simulink model "mars_rover_test_harness_chassis"  (R2025a)
settings: Solver=ode23t  StartTime=0.0  StopTime=30  FixedStep=1e-10  MaxStep=1e-1  RelTol=1e-3  AbsTol=1e-3  EnableMultiTasking=on
undefined symbols (not defined in the file): arm_q0, Control, L1, L2, L3, LS1, LS3, R1, R2, R3, Rover, RS1, RS3, X, Y, Z
libraries: sm_lib x119, nesl_utility x99, fl_lib x85, sdl_lib x20, ee_lib x10, mars_rover_lib x8, simulink x5, slpidlib x3, batteryecm_lib x2
(part 6 of 8)

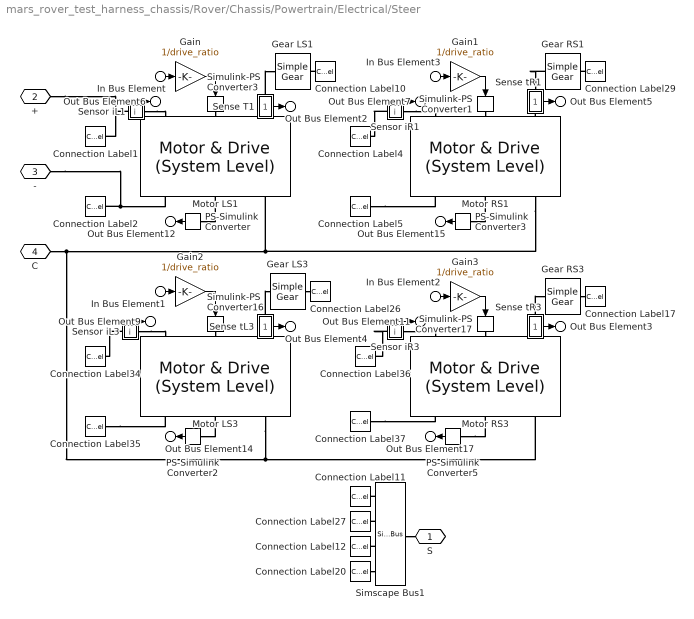
== system mars_rover_test_harness_chassis/Rover/Chassis/Powertrain/Electrical/Steer ==
  In Bus Element : Inport  PortName=Trq  Element=trq.L1
  In Bus Element1 : Inport  PortName=Trq  Element=trq.L3
  In Bus Element2 : Inport  PortName=Trq  Element=trq.R3
  In Bus Element3 : Inport  PortName=Trq  Element=trq.R1
  Connection Label{1,4,34,36} (4 alike) : ConnectionLabel  Label=p
  Connection Label10 : ConnectionLabel  Label=LS1
  Connection Label11 : ConnectionLabel  Label=LS1
  Connection Label12 : ConnectionLabel  Label=RS1
  Connection Label17 : ConnectionLabel  Label=RS3
  Connection Label{2,5,35,37} (4 alike) : ConnectionLabel  Label=n
  Connection Label20 : ConnectionLabel  Label=RS3
  Connection Label26 : ConnectionLabel  Label=LS3
  Connection Label27 : ConnectionLabel  Label=LS3
  Connection Label29 : ConnectionLabel  Label=RS1
  Gain{,1..3} (4 alike) : Gain  Gain=1/drive_ratio
  Gear LS3 : sdl_lib/Gears/Simple Gear  ratio=drive_ratio  rotation_direction=sdl.enum.shaftOutputDirection.same  friction_model=sdl.enum.gear_efficiencies_load.off  T_noload=0.1 N*m  T_nom=5 N*m  efficiency_nom=0.8  efficiency=drive_efficiency  temperature_TLU=[280, 300, 320] K  load_TLU=[1, 5, 10] N*m  efficiency_TLU=[.95, .9, .85]  efficiency_TLU2=[.85, .8, .75; .95, .9, .85; .85, .8, .7]  w_thr=0.01 rad/s  pwr_thr=0.001 W  enable_backlash=false  hardstop_model=simscape.enum.hardstop.smooth  backlash_distance=1e-3 mm  r_base=0.1 m  transition=1e-4 mm  backlash_stiffness=1e7 N/m  backlash_damping=1e6 N/(m/s)  coeff_rest=0  v_tol=0.001 m/s  f_tol=0 N  mu_visc=[0, 0] N*m/(rad/s)  thermal_mass=50 J/K  temperature_specify=off  temperature_priority=High  temperature=300 K  temperature_nominal_specify=off  temperature_nominal_value=1  temperature_nominal_unit=K  x_backlash_specify=off  x_backlash_priority=None  x_backlash=0 mm  x_backlash_nominal_specify=off  x_backlash_nominal_value=1  x_backlash_nominal_unit=mm  f_hardstop_specify=off  f_hardstop_priority=None  f_hardstop=0 N  f_hardstop_nominal_specify=off  f_hardstop_nominal_value=1  f_hardstop_nominal_unit=N  v_backlash_specify=off  v_backlash_priority=None  v_backlash=0 m/s  v_backlash_nominal_specify=off  v_backlash_nominal_value=1  v_backlash_nominal_unit=m/s
  Gear RS1 : sdl_lib/Gears/Simple Gear  ratio=drive_ratio  rotation_direction=sdl.enum.shaftOutputDirection.same  friction_model=sdl.enum.gear_efficiencies_load.off  T_noload=0.1 N*m  T_nom=5 N*m  efficiency_nom=0.8  efficiency=drive_efficiency  temperature_TLU=[280, 300, 320] K  load_TLU=[1, 5, 10] N*m  efficiency_TLU=[.95, .9, .85]  efficiency_TLU2=[.85, .8, .75; .95, .9, .85; .85, .8, .7]  w_thr=0.01 rad/s  pwr_thr=0.001 W  enable_backlash=false  hardstop_model=simscape.enum.hardstop.smooth  backlash_distance=1e-3 mm  r_base=0.1 m  transition=1e-4 mm  backlash_stiffness=1e7 N/m  backlash_damping=1e6 N/(m/s)  coeff_rest=0  v_tol=0.001 m/s  f_tol=0 N  mu_visc=[0, 0] N*m/(rad/s)  thermal_mass=50 J/K  temperature_specify=off  temperature_priority=High  temperature=300 K  temperature_nominal_specify=off  temperature_nominal_value=1  temperature_nominal_unit=K  x_backlash_specify=off  x_backlash_priority=None  x_backlash=0 mm  x_backlash_nominal_specify=off  x_backlash_nominal_value=1  x_backlash_nominal_unit=mm  f_hardstop_specify=off  f_hardstop_priority=None  f_hardstop=0 N  f_hardstop_nominal_specify=off  f_hardstop_nominal_value=1  f_hardstop_nominal_unit=N  v_backlash_specify=off  v_backlash_priority=None  v_backlash=0 m/s  v_backlash_nominal_specify=off  v_backlash_nominal_value=1  v_backlash_nominal_unit=m/s
  Gear RS3 : sdl_lib/Gears/Simple Gear  ratio=drive_ratio  rotation_direction=sdl.enum.shaftOutputDirection.same  friction_model=sdl.enum.gear_efficiencies_load.off  T_noload=0.1 N*m  T_nom=5 N*m  efficiency_nom=0.8  efficiency=drive_efficiency  temperature_TLU=[280, 300, 320] K  load_TLU=[1, 5, 10] N*m  efficiency_TLU=[.95, .9, .85]  efficiency_TLU2=[.85, .8, .75; .95, .9, .85; .85, .8, .7]  w_thr=0.01 rad/s  pwr_thr=0.001 W  enable_backlash=false  hardstop_model=simscape.enum.hardstop.smooth  backlash_distance=1e-3 mm  r_base=0.1 m  transition=1e-4 mm  backlash_stiffness=1e7 N/m  backlash_damping=1e6 N/(m/s)  coeff_rest=0  v_tol=0.001 m/s  f_tol=0 N  mu_visc=[0, 0] N*m/(rad/s)  thermal_mass=50 J/K  temperature_specify=off  temperature_priority=High  temperature=300 K  temperature_nominal_specify=off  temperature_nominal_value=1  temperature_nominal_unit=K  x_backlash_specify=off  x_backlash_priority=None  x_backlash=0 mm  x_backlash_nominal_specify=off  x_backlash_nominal_value=1  x_backlash_nominal_unit=mm  f_hardstop_specify=off  f_hardstop_priority=None  f_hardstop=0 N  f_hardstop_nominal_specify=off  f_hardstop_nominal_value=1  f_hardstop_nominal_unit=N  v_backlash_specify=off  v_backlash_priority=None  v_backlash=0 m/s  v_backlash_nominal_specify=off  v_backlash_nominal_value=1  v_backlash_nominal_unit=m/s
  Gear LS1 : sdl_lib/Gears/Simple Gear  ratio=drive_ratio  rotation_direction=sdl.enum.shaftOutputDirection.same  friction_model=sdl.enum.gear_efficiencies_load.off  T_noload=0.1 N*m  T_nom=5 N*m  efficiency_nom=0.8  efficiency=drive_efficiency  temperature_TLU=[280, 300, 320] K  load_TLU=[1, 5, 10] N*m  efficiency_TLU=[.95, .9, .85]  efficiency_TLU2=[.85, .8, .75; .95, .9, .85; .85, .8, .7]  w_thr=0.01 rad/s  pwr_thr=0.001 W  enable_backlash=false  hardstop_model=simscape.enum.hardstop.smooth  backlash_distance=1e-3 mm  r_base=0.1 m  transition=1e-4 mm  backlash_stiffness=1e7 N/m  backlash_damping=1e6 N/(m/s)  coeff_rest=0  v_tol=0.001 m/s  f_tol=0 N  mu_visc=[0, 0] N*m/(rad/s)  thermal_mass=50 J/K  temperature_specify=off  temperature_priority=High  temperature=300 K  temperature_nominal_specify=off  temperature_nominal_value=1  temperature_nominal_unit=K  x_backlash_specify=off  x_backlash_priority=None  x_backlash=0 mm  x_backlash_nominal_specify=off  x_backlash_nominal_value=1  x_backlash_nominal_unit=mm  f_hardstop_specify=off  f_hardstop_priority=None  f_hardstop=0 N  f_hardstop_nominal_specify=off  f_hardstop_nominal_value=1  f_hardstop_nominal_unit=N  v_backlash_specify=off  v_backlash_priority=None  v_backlash=0 m/s  v_backlash_nominal_specify=off  v_backlash_nominal_value=1  v_backlash_nominal_unit=m/s
  Motor LS1 : ee_lib/Electromechanical/Motor & Drive (System Level)  torque_speed_param=ee.enum.electromech.envelope.torque_power  overtorque_param=ee.enum.electromech.overtorque.no  T_t=[.09, .08, .07, 0] N*m  T_t_intermittent=[.36, .32, .28, 0] N*m  T_t_2D=[.09, .09, .09; .08, .08, .08; .07, .07, .07; 0, 0, 0] N*m  T_t_intermittent_2D=[.36, .36, .36; .32, .32, .32; .28, .28, .28; 0, 0, 0] N*m  w_t=[0, 3750, 7500, 8000] rpm  vdc_t=[6, 12, 24] V  torque_max=trq_max N*m  power_max=power_max W  torque_max_intermittent=0.4 N*m  power_max_intermittent=120 W  time_overtorque=30 s  time_recover=60 s  Tc=trq_tc s  EnableSwitch=simscape.enum.onoff.off  losses_param=1  eff=eff_overall  w_eff=eff_spd rpm  T_eff=eff_trq N*m  Piron=0 % not important in first iteration W  Pbase=0 % not important in first iteration W  w_eff_vec=[-8000, -4000, 0, 4000, 8000] rpm  T_eff_vec=[0, .03, .06, .09] N*m  v_eff_vec=[100, 250, 400] V  losses_mat=[1.49, 1.67, 2.21, 3.1; .42, .69, 1.14, 2.03; .06, .24, .78, 1.68; .42, .69, 1.14, 2.03; 1.49, 1.67, 2.21, 3.1] W  efficiency_mat=[95, 95, 95, 95; 95, 95, 95, 95; 95, 95, 95, 95; 95, 95, 95, 95; 95, 95, 95, 95]  losses_mat_3D=ones(5, 4, 3) W  efficiency_mat_3D=95 * ones(5, 4, 3)  Res=0 % not important in first iteration Ohm  J=0 kg*m^2  lam=rotor_d N*m/(rad/s)  speed0=0 rpm  faulted_specify=off  faulted_priority=None  faulted=0  faulted_nominal_specify=off  faulted_nominal_value=1  faulted_nominal_unit=1  isSwitchedOff_specify=off  isSwitchedOff_priority=None  isSwitchedOff=0  isSwitchedOff_nominal_specify=off  isSwitchedOff_nominal_value=1  isSwitchedOff_nominal_unit=1  torqueLimitContinuous_specify=off  torqueLimitContinuous_priority=None  torqueLimitContinuous=0 N*m  torqueLimitContinuous_nominal_specify=off  torqueLimitContinuous_nominal_value=1  torqueLimitContinuous_nominal_unit=N*m  alpha=3.93e-3 1/K  Tmeas=25 degC  Tmeas2=125 degC  losses_mat_T2=[1.49, 1.74, 2.49, 3.74; .42, .67, 1.42, 2.67; .06, .31, 1.06, 2.31; .42, .67, 1.42, 2.67; 1.49, 1.74, 2.49, 3.74] W  efficiency_mat_T2=[95, 95, 95, 95; 95, 95, 95, 95; 95, 95, 95, 95; 95, 95, 95, 95; 95, 95, 95, 95]  losses_mat_3D_T2=ones(5, 4, 3) W  efficiency_mat_3D_T2=95 * ones(5, 4, 3)  thermal_mass=100 J/K  initial_temperature=25 degC
  Motor LS3 : ee_lib/Electromechanical/Motor & Drive (System Level)  torque_speed_param=ee.enum.electromech.envelope.torque_power  overtorque_param=ee.enum.electromech.overtorque.no  T_t=[.09, .08, .07, 0] N*m  T_t_intermittent=[.36, .32, .28, 0] N*m  T_t_2D=[.09, .09, .09; .08, .08, .08; .07, .07, .07; 0, 0, 0] N*m  T_t_intermittent_2D=[.36, .36, .36; .32, .32, .32; .28, .28, .28; 0, 0, 0] N*m  w_t=[0, 3750, 7500, 8000] rpm  vdc_t=[6, 12, 24] V  torque_max=trq_max N*m  power_max=power_max W  torque_max_intermittent=0.4 N*m  power_max_intermittent=120 W  time_overtorque=30 s  time_recover=60 s  Tc=trq_tc s  EnableSwitch=simscape.enum.onoff.off  losses_param=1  eff=eff_overall  w_eff=eff_spd rpm  T_eff=eff_trq N*m  Piron=0 % not important in first iteration W  Pbase=0 % not important in first iteration W  w_eff_vec=[-8000, -4000, 0, 4000, 8000] rpm  T_eff_vec=[0, .03, .06, .09] N*m  v_eff_vec=[100, 250, 400] V  losses_mat=[1.49, 1.67, 2.21, 3.1; .42, .69, 1.14, 2.03; .06, .24, .78, 1.68; .42, .69, 1.14, 2.03; 1.49, 1.67, 2.21, 3.1] W  efficiency_mat=[95, 95, 95, 95; 95, 95, 95, 95; 95, 95, 95, 95; 95, 95, 95, 95; 95, 95, 95, 95]  losses_mat_3D=ones(5, 4, 3) W  efficiency_mat_3D=95 * ones(5, 4, 3)  Res=0 % not important in first iteration Ohm  J=0 kg*m^2  lam=rotor_d N*m/(rad/s)  speed0=0 rpm  faulted_specify=off  faulted_priority=None  faulted=0  faulted_nominal_specify=off  faulted_nominal_value=1  faulted_nominal_unit=1  isSwitchedOff_specify=off  isSwitchedOff_priority=None  isSwitchedOff=0  isSwitchedOff_nominal_specify=off  isSwitchedOff_nominal_value=1  isSwitchedOff_nominal_unit=1  torqueLimitContinuous_specify=off  torqueLimitContinuous_priority=None  torqueLimitContinuous=0 N*m  torqueLimitContinuous_nominal_specify=off  torqueLimitContinuous_nominal_value=1  torqueLimitContinuous_nominal_unit=N*m  alpha=3.93e-3 1/K  Tmeas=25 degC  Tmeas2=125 degC  losses_mat_T2=[1.49, 1.74, 2.49, 3.74; .42, .67, 1.42, 2.67; .06, .31, 1.06, 2.31; .42, .67, 1.42, 2.67; 1.49, 1.74, 2.49, 3.74] W  efficiency_mat_T2=[95, 95, 95, 95; 95, 95, 95, 95; 95, 95, 95, 95; 95, 95, 95, 95; 95, 95, 95, 95]  losses_mat_3D_T2=ones(5, 4, 3) W  efficiency_mat_3D_T2=95 * ones(5, 4, 3)  thermal_mass=100 J/K  initial_temperature=25 degC
  Motor RS1 : ee_lib/Electromechanical/Motor & Drive (System Level)  torque_speed_param=ee.enum.electromech.envelope.torque_power  overtorque_param=ee.enum.electromech.overtorque.no  T_t=[.09, .08, .07, 0] N*m  T_t_intermittent=[.36, .32, .28, 0] N*m  T_t_2D=[.09, .09, .09; .08, .08, .08; .07, .07, .07; 0, 0, 0] N*m  T_t_intermittent_2D=[.36, .36, .36; .32, .32, .32; .28, .28, .28; 0, 0, 0] N*m  w_t=[0, 3750, 7500, 8000] rpm  vdc_t=[6, 12, 24] V  torque_max=trq_max N*m  power_max=power_max W  torque_max_intermittent=0.4 N*m  power_max_intermittent=120 W  time_overtorque=30 s  time_recover=60 s  Tc=trq_tc s  EnableSwitch=simscape.enum.onoff.off  losses_param=1  eff=eff_overall  w_eff=eff_spd rpm  T_eff=eff_trq N*m  Piron=0 % not important in first iteration W  Pbase=0 % not important in first iteration W  w_eff_vec=[-8000, -4000, 0, 4000, 8000] rpm  T_eff_vec=[0, .03, .06, .09] N*m  v_eff_vec=[100, 250, 400] V  losses_mat=[1.49, 1.67, 2.21, 3.1; .42, .69, 1.14, 2.03; .06, .24, .78, 1.68; .42, .69, 1.14, 2.03; 1.49, 1.67, 2.21, 3.1] W  efficiency_mat=[95, 95, 95, 95; 95, 95, 95, 95; 95, 95, 95, 95; 95, 95, 95, 95; 95, 95, 95, 95]  losses_mat_3D=ones(5, 4, 3) W  efficiency_mat_3D=95 * ones(5, 4, 3)  Res=0 % not important in first iteration Ohm  J=0 kg*m^2  lam=rotor_d N*m/(rad/s)  speed0=0 rpm  faulted_specify=off  faulted_priority=None  faulted=0  faulted_nominal_specify=off  faulted_nominal_value=1  faulted_nominal_unit=1  isSwitchedOff_specify=off  isSwitchedOff_priority=None  isSwitchedOff=0  isSwitchedOff_nominal_specify=off  isSwitchedOff_nominal_value=1  isSwitchedOff_nominal_unit=1  torqueLimitContinuous_specify=off  torqueLimitContinuous_priority=None  torqueLimitContinuous=0 N*m  torqueLimitContinuous_nominal_specify=off  torqueLimitContinuous_nominal_value=1  torqueLimitContinuous_nominal_unit=N*m  alpha=3.93e-3 1/K  Tmeas=25 degC  Tmeas2=125 degC  losses_mat_T2=[1.49, 1.74, 2.49, 3.74; .42, .67, 1.42, 2.67; .06, .31, 1.06, 2.31; .42, .67, 1.42, 2.67; 1.49, 1.74, 2.49, 3.74] W  efficiency_mat_T2=[95, 95, 95, 95; 95, 95, 95, 95; 95, 95, 95, 95; 95, 95, 95, 95; 95, 95, 95, 95]  losses_mat_3D_T2=ones(5, 4, 3) W  efficiency_mat_3D_T2=95 * ones(5, 4, 3)  thermal_mass=100 J/K  initial_temperature=25 degC
  Motor RS3 : ee_lib/Electromechanical/Motor & Drive (System Level)  torque_speed_param=ee.enum.electromech.envelope.torque_power  overtorque_param=ee.enum.electromech.overtorque.no  T_t=[.09, .08, .07, 0] N*m  T_t_intermittent=[.36, .32, .28, 0] N*m  T_t_2D=[.09, .09, .09; .08, .08, .08; .07, .07, .07; 0, 0, 0] N*m  T_t_intermittent_2D=[.36, .36, .36; .32, .32, .32; .28, .28, .28; 0, 0, 0] N*m  w_t=[0, 3750, 7500, 8000] rpm  vdc_t=[6, 12, 24] V  torque_max=trq_max N*m  power_max=power_max W  torque_max_intermittent=0.4 N*m  power_max_intermittent=120 W  time_overtorque=30 s  time_recover=60 s  Tc=trq_tc s  EnableSwitch=simscape.enum.onoff.off  losses_param=1  eff=eff_overall  w_eff=eff_spd rpm  T_eff=eff_trq N*m  Piron=0 % not important in first iteration W  Pbase=0 % not important in first iteration W  w_eff_vec=[-8000, -4000, 0, 4000, 8000] rpm  T_eff_vec=[0, .03, .06, .09] N*m  v_eff_vec=[100, 250, 400] V  losses_mat=[1.49, 1.67, 2.21, 3.1; .42, .69, 1.14, 2.03; .06, .24, .78, 1.68; .42, .69, 1.14, 2.03; 1.49, 1.67, 2.21, 3.1] W  efficiency_mat=[95, 95, 95, 95; 95, 95, 95, 95; 95, 95, 95, 95; 95, 95, 95, 95; 95, 95, 95, 95]  losses_mat_3D=ones(5, 4, 3) W  efficiency_mat_3D=95 * ones(5, 4, 3)  Res=0 % not important in first iteration Ohm  J=0 kg*m^2  lam=rotor_d N*m/(rad/s)  speed0=0 rpm  faulted_specify=off  faulted_priority=None  faulted=0  faulted_nominal_specify=off  faulted_nominal_value=1  faulted_nominal_unit=1  isSwitchedOff_specify=off  isSwitchedOff_priority=None  isSwitchedOff=0  isSwitchedOff_nominal_specify=off  isSwitchedOff_nominal_value=1  isSwitchedOff_nominal_unit=1  torqueLimitContinuous_specify=off  torqueLimitContinuous_priority=None  torqueLimitContinuous=0 N*m  torqueLimitContinuous_nominal_specify=off  torqueLimitContinuous_nominal_value=1  torqueLimitContinuous_nominal_unit=N*m  alpha=3.93e-3 1/K  Tmeas=25 degC  Tmeas2=125 degC  losses_mat_T2=[1.49, 1.74, 2.49, 3.74; .42, .67, 1.42, 2.67; .06, .31, 1.06, 2.31; .42, .67, 1.42, 2.67; 1.49, 1.74, 2.49, 3.74] W  efficiency_mat_T2=[95, 95, 95, 95; 95, 95, 95, 95; 95, 95, 95, 95; 95, 95, 95, 95; 95, 95, 95, 95]  losses_mat_3D_T2=ones(5, 4, 3) W  efficiency_mat_3D_T2=95 * ones(5, 4, 3)  thermal_mass=100 J/K  initial_temperature=25 degC
  PS-Simulink Converter{,2..3,5} (4 alike) : nesl_utility/PS-Simulink Converter  PhysicalDomain=network_engine_domain  SubClassName=ps_output  LeftPortType=input  RightPortType=output  PseudoPeriodic=off  Frequencies=[]  VectorFormat=1-D array  Unit=inherit  AffineConversion=off
  Sense T1 : Subsystem
      settings: PortSchema="{\"entries\":[{\"content\":{\"sides\":[{\"content\":{\"connectorIds\":[\"LConn1\"]},\"type\":\"ConnectorPlacement.EquallySpacedRectSide\",\"uuid\":\"592cc1a1-656f-47ce-ad3a-4b4dc1070b5c\"},{\"content\":{\"connectorIds\":[\"RConn1\"],\"side\":\"RIGHT\"},\"type\":\"ConnectorPlacement.EquallySpacedRectSide\",\"uuid\":\"9bca39c3-eeb4-4456-9b97-61ec2f027d42\"},{\"content\":{\"connectorIds\":[\"Out1\"],\"side\":\"TOP\"},\"type\":\"ConnectorPlacement.EquallySpacedRectSide\",\"uuid\":\"1e04bf27-fb0c-4be4-96d5-7a7c6152a7df\"}]},\"type\":\"ConnectorPlacement.EquallySpacedConnector\",\"uuid\":\"70eba8cc-e966-48e4-a1ce-5ccb9693dc60\"}],\"packageUris\":[\"http://schema.mathworks.com/mf0/Connector/R2020b\"],\"version\":\"1.0\"}"
      mask Display: disp('t')
  Sense tL3 : Subsystem
      settings: PortSchema="{\"entries\":[{\"content\":{\"sides\":[{\"content\":{\"connectorIds\":[\"LConn1\"]},\"type\":\"ConnectorPlacement.EquallySpacedRectSide\",\"uuid\":\"592cc1a1-656f-47ce-ad3a-4b4dc1070b5c\"},{\"content\":{\"connectorIds\":[\"RConn1\"],\"side\":\"RIGHT\"},\"type\":\"ConnectorPlacement.EquallySpacedRectSide\",\"uuid\":\"9bca39c3-eeb4-4456-9b97-61ec2f027d42\"},{\"content\":{\"connectorIds\":[\"Out1\"],\"side\":\"TOP\"},\"type\":\"ConnectorPlacement.EquallySpacedRectSide\",\"uuid\":\"1e04bf27-fb0c-4be4-96d5-7a7c6152a7df\"}]},\"type\":\"ConnectorPlacement.EquallySpacedConnector\",\"uuid\":\"70eba8cc-e966-48e4-a1ce-5ccb9693dc60\"}],\"packageUris\":[\"http://schema.mathworks.com/mf0/Connector/R2020b\"],\"version\":\"1.0\"}"
      mask Display: disp('t')
  Sense tR1 : Subsystem
      settings: PortSchema="{\"entries\":[{\"content\":{\"sides\":[{\"content\":{\"connectorIds\":[\"LConn1\"]},\"type\":\"ConnectorPlacement.EquallySpacedRectSide\",\"uuid\":\"592cc1a1-656f-47ce-ad3a-4b4dc1070b5c\"},{\"content\":{\"connectorIds\":[\"RConn1\"],\"side\":\"RIGHT\"},\"type\":\"ConnectorPlacement.EquallySpacedRectSide\",\"uuid\":\"9bca39c3-eeb4-4456-9b97-61ec2f027d42\"},{\"content\":{\"connectorIds\":[\"Out1\"],\"side\":\"TOP\"},\"type\":\"ConnectorPlacement.EquallySpacedRectSide\",\"uuid\":\"1e04bf27-fb0c-4be4-96d5-7a7c6152a7df\"}]},\"type\":\"ConnectorPlacement.EquallySpacedConnector\",\"uuid\":\"70eba8cc-e966-48e4-a1ce-5ccb9693dc60\"}],\"packageUris\":[\"http://schema.mathworks.com/mf0/Connector/R2020b\"],\"version\":\"1.0\"}"
      mask Display: disp('t')
  Sense tR3 : Subsystem
      settings: PortSchema="{\"entries\":[{\"content\":{\"sides\":[{\"content\":{\"connectorIds\":[\"LConn1\"]},\"type\":\"ConnectorPlacement.EquallySpacedRectSide\",\"uuid\":\"592cc1a1-656f-47ce-ad3a-4b4dc1070b5c\"},{\"content\":{\"connectorIds\":[\"RConn1\"],\"side\":\"RIGHT\"},\"type\":\"ConnectorPlacement.EquallySpacedRectSide\",\"uuid\":\"9bca39c3-eeb4-4456-9b97-61ec2f027d42\"},{\"content\":{\"connectorIds\":[\"Out1\"],\"side\":\"TOP\"},\"type\":\"ConnectorPlacement.EquallySpacedRectSide\",\"uuid\":\"1e04bf27-fb0c-4be4-96d5-7a7c6152a7df\"}]},\"type\":\"ConnectorPlacement.EquallySpacedConnector\",\"uuid\":\"70eba8cc-e966-48e4-a1ce-5ccb9693dc60\"}],\"packageUris\":[\"http://schema.mathworks.com/mf0/Connector/R2020b\"],\"version\":\"1.0\"}"
      mask Display: disp('t')
  Sensor iL1 : Subsystem
      settings: PortSchema="{\"entries\":[{\"content\":{\"sides\":[{\"content\":{\"connectorIds\":[\"LConn1\"]},\"type\":\"ConnectorPlacement.EquallySpacedRectSide\",\"uuid\":\"592cc1a1-656f-47ce-ad3a-4b4dc1070b5c\"},{\"content\":{\"connectorIds\":[\"RConn1\"],\"side\":\"RIGHT\"},\"type\":\"ConnectorPlacement.EquallySpacedRectSide\",\"uuid\":\"9bca39c3-eeb4-4456-9b97-61ec2f027d42\"},{\"content\":{\"connectorIds\":[\"Out1\"],\"side\":\"TOP\"},\"type\":\"ConnectorPlacement.EquallySpacedRectSide\",\"uuid\":\"1e04bf27-fb0c-4be4-96d5-7a7c6152a7df\"}]},\"type\":\"ConnectorPlacement.EquallySpacedConnector\",\"uuid\":\"70eba8cc-e966-48e4-a1ce-5ccb9693dc60\"}],\"packageUris\":[\"http://schema.mathworks.com/mf0/Connector/R2020b\"],\"version\":\"1.0\"}"
      mask Display: disp('i');
  Sensor iL3 : Subsystem
      settings: PortSchema="{\"entries\":[{\"content\":{\"sides\":[{\"content\":{\"connectorIds\":[\"LConn1\"]},\"type\":\"ConnectorPlacement.EquallySpacedRectSide\",\"uuid\":\"592cc1a1-656f-47ce-ad3a-4b4dc1070b5c\"},{\"content\":{\"connectorIds\":[\"RConn1\"],\"side\":\"RIGHT\"},\"type\":\"ConnectorPlacement.EquallySpacedRectSide\",\"uuid\":\"9bca39c3-eeb4-4456-9b97-61ec2f027d42\"},{\"content\":{\"connectorIds\":[\"Out1\"],\"side\":\"TOP\"},\"type\":\"ConnectorPlacement.EquallySpacedRectSide\",\"uuid\":\"1e04bf27-fb0c-4be4-96d5-7a7c6152a7df\"}]},\"type\":\"ConnectorPlacement.EquallySpacedConnector\",\"uuid\":\"70eba8cc-e966-48e4-a1ce-5ccb9693dc60\"}],\"packageUris\":[\"http://schema.mathworks.com/mf0/Connector/R2020b\"],\"version\":\"1.0\"}"
      mask Display: disp('i');
  Sensor iR1 : Subsystem
      settings: PortSchema="{\"entries\":[{\"content\":{\"sides\":[{\"content\":{\"connectorIds\":[\"LConn1\"]},\"type\":\"ConnectorPlacement.EquallySpacedRectSide\",\"uuid\":\"592cc1a1-656f-47ce-ad3a-4b4dc1070b5c\"},{\"content\":{\"connectorIds\":[\"RConn1\"],\"side\":\"RIGHT\"},\"type\":\"ConnectorPlacement.EquallySpacedRectSide\",\"uuid\":\"9bca39c3-eeb4-4456-9b97-61ec2f027d42\"},{\"content\":{\"connectorIds\":[\"Out1\"],\"side\":\"TOP\"},\"type\":\"ConnectorPlacement.EquallySpacedRectSide\",\"uuid\":\"1e04bf27-fb0c-4be4-96d5-7a7c6152a7df\"}]},\"type\":\"ConnectorPlacement.EquallySpacedConnector\",\"uuid\":\"70eba8cc-e966-48e4-a1ce-5ccb9693dc60\"}],\"packageUris\":[\"http://schema.mathworks.com/mf0/Connector/R2020b\"],\"version\":\"1.0\"}"
      mask Display: disp('i');
  Sensor iR3 : Subsystem
      settings: PortSchema="{\"entries\":[{\"content\":{\"sides\":[{\"content\":{\"connectorIds\":[\"LConn1\"]},\"type\":\"ConnectorPlacement.EquallySpacedRectSide\",\"uuid\":\"592cc1a1-656f-47ce-ad3a-4b4dc1070b5c\"},{\"content\":{\"connectorIds\":[\"RConn1\"],\"side\":\"RIGHT\"},\"type\":\"ConnectorPlacement.EquallySpacedRectSide\",\"uuid\":\"9bca39c3-eeb4-4456-9b97-61ec2f027d42\"},{\"content\":{\"connectorIds\":[\"Out1\"],\"side\":\"TOP\"},\"type\":\"ConnectorPlacement.EquallySpacedRectSide\",\"uuid\":\"1e04bf27-fb0c-4be4-96d5-7a7c6152a7df\"}]},\"type\":\"ConnectorPlacement.EquallySpacedConnector\",\"uuid\":\"70eba8cc-e966-48e4-a1ce-5ccb9693dc60\"}],\"packageUris\":[\"http://schema.mathworks.com/mf0/Connector/R2020b\"],\"version\":\"1.0\"}"
      mask Display: disp('i');
  Simscape Bus1 : SimscapeBus  HierarchyStrings=LS1;LS3;RS1;RS3
  Simulink-PS Converter{1,3,16..17} (4 alike) : nesl_utility/Simulink-PS Converter  PhysicalDomain=network_engine_domain  SubClassName=ps_input  LeftPortType=input  RightPortType=output  PseudoPeriodic=off  Frequencies=[]  NoiseDistribution=none  NoiseParameters=[]  Unit=N*m  AffineConversion=off  FilteringAndDerivatives=provide  SimscapeFilterOrder=1  InputFilterTimeConstant=0.001  UdotUserProvided=0
  S : PMIOPort  Side=Right
  + : PMIOPort  Port=2  Side=Left
  - : PMIOPort  Port=3  Side=Left
  C : PMIOPort  Port=4  Side=Right
  Out Bus Element2 : Outport  PortName=m  Element=trq.L1
  Out Bus Element4 : Outport  PortName=m  Element=trq.L3
  Out Bus Element5 : Outport  PortName=m  Element=trq.R1
  Out Bus Element3 : Outport  PortName=m  Element=trq.R3
  Out Bus Element11 : Outport  PortName=m  Element=i.R3
  Out Bus Element6 : Outport  PortName=m  Element=i.L1
  Out Bus Element9 : Outport  PortName=m  Element=i.L3
  Out Bus Element7 : Outport  PortName=m  Element=i.R1
  Out Bus Element12 : Outport  PortName=m  Element=w.L1
  Out Bus Element14 : Outport  PortName=m  Element=w.L3
  Out Bus Element15 : Outport  PortName=m  Element=w.R1
  Out Bus Element17 : Outport  PortName=m  Element=w.R3
  wires:
  Gain2/1 -> Simulink-PS Converter16/1
  In Bus Element2/1 -> Gain3/1
  In Bus Element3/1 -> Gain1/1
  In Bus Element/1 -> Gain/1
  Gain/1 -> Simulink-PS Converter3/1
  Gain1/1 -> Simulink-PS Converter1/1
  In Bus Element1/1 -> Gain2/1
  Gain3/1 -> Simulink-PS Converter17/1
  PS-Simulink Converter/1 -> Out Bus Element12/1
  Sensor iL3/1(i) -> Out Bus Element9/1
  Sense tR3/1(T) -> Out Bus Element3/1
  Sensor iR3/1(i) -> Out Bus Element11/1
  Sensor iR1/1(i) -> Out Bus Element7/1
  Sensor iL1/1(i) -> Out Bus Element6/1
  Sense tL3/1(T) -> Out Bus Element4/1
  Sense T1/1(T) -> Out Bus Element2/1
  PS-Simulink Converter5/1 -> Out Bus Element17/1
  Sense tR1/1(T) -> Out Bus Element5/1
  PS-Simulink Converter3/1 -> Out Bus Element15/1
  PS-Simulink Converter2/1 -> Out Bus Element14/1
  connections:
  Sensor iR1/RConn1 -- Motor RS1/LConn1
  Sensor iR1/LConn1 -- Connection Label4/LConn1
  Simscape Bus1/RConn1 -- S/RConn1
  Connection Label5/LConn1 -- Motor RS1/RConn1
  Motor RS1/RConn3 -- Motor LS1/RConn3 -- C/RConn1 -- Motor LS3/RConn3 -- Motor RS3/RConn3
  Connection Label37/LConn1 -- Motor RS3/RConn1
  Simulink-PS Converter3/RConn1 -- Motor LS1/LConn2
  Simulink-PS Converter16/RConn1 -- Motor LS3/LConn2
  Sensor iL3/LConn1 -- Connection Label34/LConn1
  Connection Label29/LConn1 -- Gear RS1/RConn1
  Simscape Bus1/LConn1 -- Connection Label11/LConn1
  Simulink-PS Converter17/RConn1 -- Motor RS3/LConn2
  Simscape Bus1/LConn3 -- Connection Label12/LConn1
  Simulink-PS Converter1/RConn1 -- Motor RS1/LConn2
  Simscape Bus1/LConn2 -- Connection Label27/LConn1
  Sensor iR3/RConn1 -- Motor RS3/LConn1
  Sensor iL1/RConn1 -- Motor LS1/LConn1
  Sensor iR3/LConn1 -- Connection Label36/LConn1
  PS-Simulink Converter2/LConn1 -- Motor LS3/RConn2
  Connection Label35/LConn1 -- Motor LS3/RConn1
  Sensor iL3/RConn1 -- Motor LS3/LConn1
  Connection Label20/LConn1 -- Simscape Bus1/LConn4
  PS-Simulink Converter5/LConn1 -- Motor RS3/RConn2
  PS-Simulink Converter/LConn1 -- Motor LS1/RConn2
  PS-Simulink Converter3/LConn1 -- Motor RS1/RConn2
  +/RConn1 -- Sensor iL1/LConn1 -- Connection Label1/LConn1
  -/RConn1 -- Motor LS1/RConn1 -- Connection Label2/LConn1
  Connection Label10/LConn1 -- Gear LS1/RConn1
  Gear LS3/RConn1 -- Connection Label26/LConn1
  Gear RS3/RConn1 -- Connection Label17/LConn1
  Sense T1/LConn1 -- Gear LS1/LConn1
  Sense T1/RConn1 -- Motor LS1/LConn3
  Motor RS1/LConn3 -- Sense tR1/RConn1
  Gear RS1/LConn1 -- Sense tR1/LConn1
  Sense tL3/LConn1 -- Gear LS3/LConn1
  Sense tL3/RConn1 -- Motor LS3/LConn3
  Sense tR3/LConn1 -- Gear RS3/LConn1
  Motor RS3/LConn3 -- Sense tR3/RConn1

== system mars_rover_test_harness_chassis/Rover/Chassis/Powertrain/Ideal/Calculate Power ==
  S : Inport
  D : Inport  Port=2
  Abs : Abs  ZeroCross=off  SaturateOnIntegerOverflow=off
  Bus Selector : BusSelector  OutputSignals=w.L1,trq.L1,w.L3,trq.L3,w.R1,trq.R1,w.R3,trq.R3
  Bus Selector1 : BusSelector  OutputSignals=w.L1,trq.L1,w.L2,trq.L2,w.L3,trq.L3,w.R1,trq.R1,w.R2,trq.R2,w.R3,trq.R3
  Product{,1..9} (10 alike) : Product
  R : Gain  Gain=1/100
  Sum : Sum  Inputs=++++
  Sum1 : Sum  Inputs=++++++
  Sum2 : Sum
  i : Outport
  wires:
  S/1 -> Bus Selector/1
  Bus Selector/1 -> Product/1  "<L1>"
  Bus Selector/2 -> Product/2  "<L1>"
  Bus Selector/3 -> Product1/1  "<L3>"
  Bus Selector/4 -> Product1/2  "<L3>"
  Bus Selector/6 -> Product2/2  "<R1>"
  Bus Selector/5 -> Product2/1  "<R1>"
  Product/1 -> Sum/1
  Product1/1 -> Sum/2
  Product2/1 -> Sum/3
  Product3/1 -> Sum/4
  D/1 -> Bus Selector1/1
  Product7/1 -> Sum1/4
  Product6/1 -> Sum1/3
  Product5/1 -> Sum1/2
  Product4/1 -> Sum1/1
  Bus Selector1/1 -> Product4/1  "<L1>"
  Bus Selector1/2 -> Product4/2  "<L1>"
  Product8/1 -> Sum1/5
  Product9/1 -> Sum1/6
  Bus Selector1/3 -> Product5/1  "<L2>"
  Bus Selector1/4 -> Product5/2  "<L2>"
  Bus Selector1/5 -> Product6/1  "<L3>"
  Bus Selector1/6 -> Product6/2  "<L3>"
  Bus Selector1/7 -> Product7/1  "<R1>"
  Bus Selector1/8 -> Product7/2  "<R1>"
  Bus Selector1/9 -> Product8/1  "<R2>"
  Bus Selector1/10 -> Product8/2  "<R2>"
  Bus Selector1/11 -> Product9/1  "<R3>"
  Bus Selector1/12 -> Product9/2  "<R3>"
  Sum1/1 -> Sum2/2
  Sum/1 -> Sum2/1
  Sum2/1 -> Abs/1
  Abs/1 -> R/1
  Bus Selector/7 -> Product3/1  "<R3>"
  Bus Selector/8 -> Product3/2  "<R3>"
  R/1 -> i/1

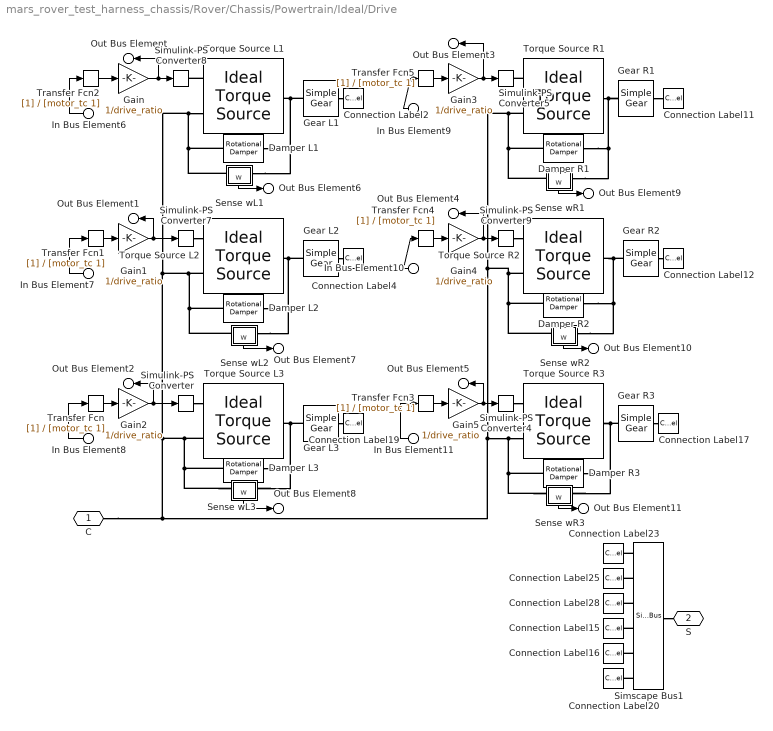
== system mars_rover_test_harness_chassis/Rover/Chassis/Powertrain/Ideal/Drive ==
  In Bus Element6 : Inport  PortName=Trq  Element=trq.L1
  In Bus Element7 : Inport  PortName=Trq  Element=trq.L2
  In Bus Element8 : Inport  PortName=Trq  Element=trq.L3
  In Bus Element9 : Inport  PortName=Trq  Element=trq.R1
  In Bus Element10 : Inport  PortName=Trq  Element=trq.R2
  In Bus Element11 : Inport  PortName=Trq  Element=trq.R3
  Connection Label11 : ConnectionLabel  Label=R1
  Connection Label12 : ConnectionLabel  Label=R2
  Connection Label15 : ConnectionLabel  Label=R1
  Connection Label16 : ConnectionLabel  Label=R2
  Connection Label17 : ConnectionLabel  Label=R3
  Connection Label19 : ConnectionLabel  Label=L3
  Connection Label2 : ConnectionLabel  Label=L1
  Connection Label20 : ConnectionLabel  Label=R3
  Connection Label23 : ConnectionLabel  Label=L1
  Connection Label25 : ConnectionLabel  Label=L2
  Connection Label28 : ConnectionLabel  Label=L3
  Connection Label4 : ConnectionLabel  Label=L2
  Damper L1 : fl_lib/Mechanical/Rotational Elements/Rotational Damper  D=motor_d N*m/(rad/s)  w_specify=off  w_priority=None  w=0 rad/s  w_nominal_specify=off  w_nominal_value=1  w_nominal_unit=rad/s  t_specify=off  t_priority=None  t=0 N*m  t_nominal_specify=off  t_nominal_value=1  t_nominal_unit=N*m
  Damper L2 : fl_lib/Mechanical/Rotational Elements/Rotational Damper  D=motor_d N*m/(rad/s)  w_specify=off  w_priority=None  w=0 rad/s  w_nominal_specify=off  w_nominal_value=1  w_nominal_unit=rad/s  t_specify=off  t_priority=None  t=0 N*m  t_nominal_specify=off  t_nominal_value=1  t_nominal_unit=N*m
  Damper L3 : fl_lib/Mechanical/Rotational Elements/Rotational Damper  D=motor_d N*m/(rad/s)  w_specify=off  w_priority=None  w=0 rad/s  w_nominal_specify=off  w_nominal_value=1  w_nominal_unit=rad/s  t_specify=off  t_priority=None  t=0 N*m  t_nominal_specify=off  t_nominal_value=1  t_nominal_unit=N*m
  Damper R1 : fl_lib/Mechanical/Rotational Elements/Rotational Damper  D=motor_d N*m/(rad/s)  w_specify=off  w_priority=None  w=0 rad/s  w_nominal_specify=off  w_nominal_value=1  w_nominal_unit=rad/s  t_specify=off  t_priority=None  t=0 N*m  t_nominal_specify=off  t_nominal_value=1  t_nominal_unit=N*m
  Damper R2 : fl_lib/Mechanical/Rotational Elements/Rotational Damper  D=motor_d N*m/(rad/s)  w_specify=off  w_priority=None  w=0 rad/s  w_nominal_specify=off  w_nominal_value=1  w_nominal_unit=rad/s  t_specify=off  t_priority=None  t=0 N*m  t_nominal_specify=off  t_nominal_value=1  t_nominal_unit=N*m
  Damper R3 : fl_lib/Mechanical/Rotational Elements/Rotational Damper  D=motor_d N*m/(rad/s)  w_specify=off  w_priority=None  w=0 rad/s  w_nominal_specify=off  w_nominal_value=1  w_nominal_unit=rad/s  t_specify=off  t_priority=None  t=0 N*m  t_nominal_specify=off  t_nominal_value=1  t_nominal_unit=N*m
  Gain{,1..5} (6 alike) : Gain  Gain=1/drive_ratio
  Gear L1 : sdl_lib/Gears/Simple Gear  ratio=drive_ratio  rotation_direction=sdl.enum.shaftOutputDirection.same  friction_model=sdl.enum.gear_efficiencies_load.off  T_noload=0.1 N*m  T_nom=5 N*m  efficiency_nom=0.8  efficiency=drive_efficiency  temperature_TLU=[280, 300, 320] K  load_TLU=[1, 5, 10] N*m  efficiency_TLU=[.95, .9, .85]  efficiency_TLU2=[.85, .8, .75; .95, .9, .85; .85, .8, .7]  w_thr=0.01 rad/s  pwr_thr=0.001 W  enable_backlash=false  hardstop_model=simscape.enum.hardstop.smooth  backlash_distance=1e-3 mm  r_base=0.1 m  transition=1e-4 mm  backlash_stiffness=1e7 N/m  backlash_damping=1e6 N/(m/s)  coeff_rest=0  v_tol=0.001 m/s  f_tol=0 N  mu_visc=[0, 0] N*m/(rad/s)  thermal_mass=50 J/K  temperature_specify=off  temperature_priority=High  temperature=300 K  temperature_nominal_specify=off  temperature_nominal_value=1  temperature_nominal_unit=K  x_backlash_specify=off  x_backlash_priority=None  x_backlash=0 mm  x_backlash_nominal_specify=off  x_backlash_nominal_value=1  x_backlash_nominal_unit=mm  f_hardstop_specify=off  f_hardstop_priority=None  f_hardstop=0 N  f_hardstop_nominal_specify=off  f_hardstop_nominal_value=1  f_hardstop_nominal_unit=N  v_backlash_specify=off  v_backlash_priority=None  v_backlash=0 m/s  v_backlash_nominal_specify=off  v_backlash_nominal_value=1  v_backlash_nominal_unit=m/s
  Gear L2 : sdl_lib/Gears/Simple Gear  ratio=drive_ratio  rotation_direction=sdl.enum.shaftOutputDirection.same  friction_model=sdl.enum.gear_efficiencies_load.off  T_noload=0.1 N*m  T_nom=5 N*m  efficiency_nom=0.8  efficiency=drive_efficiency  temperature_TLU=[280, 300, 320] K  load_TLU=[1, 5, 10] N*m  efficiency_TLU=[.95, .9, .85]  efficiency_TLU2=[.85, .8, .75; .95, .9, .85; .85, .8, .7]  w_thr=0.01 rad/s  pwr_thr=0.001 W  enable_backlash=false  hardstop_model=simscape.enum.hardstop.smooth  backlash_distance=1e-3 mm  r_base=0.1 m  transition=1e-4 mm  backlash_stiffness=1e7 N/m  backlash_damping=1e6 N/(m/s)  coeff_rest=0  v_tol=0.001 m/s  f_tol=0 N  mu_visc=[0, 0] N*m/(rad/s)  thermal_mass=50 J/K  temperature_specify=off  temperature_priority=High  temperature=300 K  temperature_nominal_specify=off  temperature_nominal_value=1  temperature_nominal_unit=K  x_backlash_specify=off  x_backlash_priority=None  x_backlash=0 mm  x_backlash_nominal_specify=off  x_backlash_nominal_value=1  x_backlash_nominal_unit=mm  f_hardstop_specify=off  f_hardstop_priority=None  f_hardstop=0 N  f_hardstop_nominal_specify=off  f_hardstop_nominal_value=1  f_hardstop_nominal_unit=N  v_backlash_specify=off  v_backlash_priority=None  v_backlash=0 m/s  v_backlash_nominal_specify=off  v_backlash_nominal_value=1  v_backlash_nominal_unit=m/s
  Gear L3 : sdl_lib/Gears/Simple Gear  ratio=drive_ratio  rotation_direction=sdl.enum.shaftOutputDirection.same  friction_model=sdl.enum.gear_efficiencies_load.off  T_noload=0.1 N*m  T_nom=5 N*m  efficiency_nom=0.8  efficiency=drive_efficiency  temperature_TLU=[280, 300, 320] K  load_TLU=[1, 5, 10] N*m  efficiency_TLU=[.95, .9, .85]  efficiency_TLU2=[.85, .8, .75; .95, .9, .85; .85, .8, .7]  w_thr=0.01 rad/s  pwr_thr=0.001 W  enable_backlash=false  hardstop_model=simscape.enum.hardstop.smooth  backlash_distance=1e-3 mm  r_base=0.1 m  transition=1e-4 mm  backlash_stiffness=1e7 N/m  backlash_damping=1e6 N/(m/s)  coeff_rest=0  v_tol=0.001 m/s  f_tol=0 N  mu_visc=[0, 0] N*m/(rad/s)  thermal_mass=50 J/K  temperature_specify=off  temperature_priority=High  temperature=300 K  temperature_nominal_specify=off  temperature_nominal_value=1  temperature_nominal_unit=K  x_backlash_specify=off  x_backlash_priority=None  x_backlash=0 mm  x_backlash_nominal_specify=off  x_backlash_nominal_value=1  x_backlash_nominal_unit=mm  f_hardstop_specify=off  f_hardstop_priority=None  f_hardstop=0 N  f_hardstop_nominal_specify=off  f_hardstop_nominal_value=1  f_hardstop_nominal_unit=N  v_backlash_specify=off  v_backlash_priority=None  v_backlash=0 m/s  v_backlash_nominal_specify=off  v_backlash_nominal_value=1  v_backlash_nominal_unit=m/s
  Gear R1 : sdl_lib/Gears/Simple Gear  ratio=drive_ratio  rotation_direction=sdl.enum.shaftOutputDirection.same  friction_model=sdl.enum.gear_efficiencies_load.off  T_noload=0.1 N*m  T_nom=5 N*m  efficiency_nom=0.8  efficiency=drive_efficiency  temperature_TLU=[280, 300, 320] K  load_TLU=[1, 5, 10] N*m  efficiency_TLU=[.95, .9, .85]  efficiency_TLU2=[.85, .8, .75; .95, .9, .85; .85, .8, .7]  w_thr=0.01 rad/s  pwr_thr=0.001 W  enable_backlash=false  hardstop_model=simscape.enum.hardstop.smooth  backlash_distance=1e-3 mm  r_base=0.1 m  transition=1e-4 mm  backlash_stiffness=1e7 N/m  backlash_damping=1e6 N/(m/s)  coeff_rest=0  v_tol=0.001 m/s  f_tol=0 N  mu_visc=[0, 0] N*m/(rad/s)  thermal_mass=50 J/K  temperature_specify=off  temperature_priority=High  temperature=300 K  temperature_nominal_specify=off  temperature_nominal_value=1  temperature_nominal_unit=K  x_backlash_specify=off  x_backlash_priority=None  x_backlash=0 mm  x_backlash_nominal_specify=off  x_backlash_nominal_value=1  x_backlash_nominal_unit=mm  f_hardstop_specify=off  f_hardstop_priority=None  f_hardstop=0 N  f_hardstop_nominal_specify=off  f_hardstop_nominal_value=1  f_hardstop_nominal_unit=N  v_backlash_specify=off  v_backlash_priority=None  v_backlash=0 m/s  v_backlash_nominal_specify=off  v_backlash_nominal_value=1  v_backlash_nominal_unit=m/s
  Gear R2 : sdl_lib/Gears/Simple Gear  ratio=drive_ratio  rotation_direction=sdl.enum.shaftOutputDirection.same  friction_model=sdl.enum.gear_efficiencies_load.off  T_noload=0.1 N*m  T_nom=5 N*m  efficiency_nom=0.8  efficiency=drive_efficiency  temperature_TLU=[280, 300, 320] K  load_TLU=[1, 5, 10] N*m  efficiency_TLU=[.95, .9, .85]  efficiency_TLU2=[.85, .8, .75; .95, .9, .85; .85, .8, .7]  w_thr=0.01 rad/s  pwr_thr=0.001 W  enable_backlash=false  hardstop_model=simscape.enum.hardstop.smooth  backlash_distance=1e-3 mm  r_base=0.1 m  transition=1e-4 mm  backlash_stiffness=1e7 N/m  backlash_damping=1e6 N/(m/s)  coeff_rest=0  v_tol=0.001 m/s  f_tol=0 N  mu_visc=[0, 0] N*m/(rad/s)  thermal_mass=50 J/K  temperature_specify=off  temperature_priority=High  temperature=300 K  temperature_nominal_specify=off  temperature_nominal_value=1  temperature_nominal_unit=K  x_backlash_specify=off  x_backlash_priority=None  x_backlash=0 mm  x_backlash_nominal_specify=off  x_backlash_nominal_value=1  x_backlash_nominal_unit=mm  f_hardstop_specify=off  f_hardstop_priority=None  f_hardstop=0 N  f_hardstop_nominal_specify=off  f_hardstop_nominal_value=1  f_hardstop_nominal_unit=N  v_backlash_specify=off  v_backlash_priority=None  v_backlash=0 m/s  v_backlash_nominal_specify=off  v_backlash_nominal_value=1  v_backlash_nominal_unit=m/s
  Gear R3 : sdl_lib/Gears/Simple Gear  ratio=drive_ratio  rotation_direction=sdl.enum.shaftOutputDirection.same  friction_model=sdl.enum.gear_efficiencies_load.off  T_noload=0.1 N*m  T_nom=5 N*m  efficiency_nom=0.8  efficiency=drive_efficiency  temperature_TLU=[280, 300, 320] K  load_TLU=[1, 5, 10] N*m  efficiency_TLU=[.95, .9, .85]  efficiency_TLU2=[.85, .8, .75; .95, .9, .85; .85, .8, .7]  w_thr=0.01 rad/s  pwr_thr=0.001 W  enable_backlash=false  hardstop_model=simscape.enum.hardstop.smooth  backlash_distance=1e-3 mm  r_base=0.1 m  transition=1e-4 mm  backlash_stiffness=1e7 N/m  backlash_damping=1e6 N/(m/s)  coeff_rest=0  v_tol=0.001 m/s  f_tol=0 N  mu_visc=[0, 0] N*m/(rad/s)  thermal_mass=50 J/K  temperature_specify=off  temperature_priority=High  temperature=300 K  temperature_nominal_specify=off  temperature_nominal_value=1  temperature_nominal_unit=K  x_backlash_specify=off  x_backlash_priority=None  x_backlash=0 mm  x_backlash_nominal_specify=off  x_backlash_nominal_value=1  x_backlash_nominal_unit=mm  f_hardstop_specify=off  f_hardstop_priority=None  f_hardstop=0 N  f_hardstop_nominal_specify=off  f_hardstop_nominal_value=1  f_hardstop_nominal_unit=N  v_backlash_specify=off  v_backlash_priority=None  v_backlash=0 m/s  v_backlash_nominal_specify=off  v_backlash_nominal_value=1  v_backlash_nominal_unit=m/s
  Sense wL1 : Subsystem
      settings: PortSchema="{\"entries\":[{\"content\":{\"sides\":[{\"content\":{\"connectorIds\":[\"LConn1\"]},\"type\":\"ConnectorPlacement.EquallySpacedRectSide\",\"uuid\":\"592cc1a1-656f-47ce-ad3a-4b4dc1070b5c\"},{\"content\":{\"connectorIds\":[\"RConn1\"],\"side\":\"RIGHT\"},\"type\":\"ConnectorPlacement.EquallySpacedRectSide\",\"uuid\":\"9bca39c3-eeb4-4456-9b97-61ec2f027d42\"},{\"content\":{\"connectorIds\":[],\"side\":\"TOP\"},\"type\":\"ConnectorPlacement.EquallySpacedRectSide\",\"uuid\":\"1e04bf27-fb0c-4be4-96d5-7a7c6152a7df\"},{\"content\":{\"connectorIds\":[\"Out1\"],\"side\":\"BOTTOM\"},\"type\":\"ConnectorPlacement.EquallySpacedRectSide\",\"uuid\":\"fcca2b0e-3afa-4320-884d-439bb49264b6\"}]},\"type\":\"ConnectorPlacement.EquallySpacedConnector\",\"uuid\":\"70eba8cc-e966-48e4-a1ce-5ccb9693dc60\"}],\"packageUris\":[\"http://schema.mathworks.com/mf0/Connector/R2020b\"],\"version\":\"1.0\"}"
      mask Display: disp('w');
  Sense wL2 : Subsystem
      settings: PortSchema="{\"entries\":[{\"content\":{\"sides\":[{\"content\":{\"connectorIds\":[\"LConn1\"]},\"type\":\"ConnectorPlacement.EquallySpacedRectSide\",\"uuid\":\"592cc1a1-656f-47ce-ad3a-4b4dc1070b5c\"},{\"content\":{\"connectorIds\":[\"RConn1\"],\"side\":\"RIGHT\"},\"type\":\"ConnectorPlacement.EquallySpacedRectSide\",\"uuid\":\"9bca39c3-eeb4-4456-9b97-61ec2f027d42\"},{\"content\":{\"connectorIds\":[],\"side\":\"TOP\"},\"type\":\"ConnectorPlacement.EquallySpacedRectSide\",\"uuid\":\"1e04bf27-fb0c-4be4-96d5-7a7c6152a7df\"},{\"content\":{\"connectorIds\":[\"Out1\"],\"side\":\"BOTTOM\"},\"type\":\"ConnectorPlacement.EquallySpacedRectSide\",\"uuid\":\"fcca2b0e-3afa-4320-884d-439bb49264b6\"}]},\"type\":\"ConnectorPlacement.EquallySpacedConnector\",\"uuid\":\"70eba8cc-e966-48e4-a1ce-5ccb9693dc60\"}],\"packageUris\":[\"http://schema.mathworks.com/mf0/Connector/R2020b\"],\"version\":\"1.0\"}"
      mask Display: disp('w');
  Sense wL3 : Subsystem
      settings: PortSchema="{\"entries\":[{\"content\":{\"sides\":[{\"content\":{\"connectorIds\":[\"LConn1\"]},\"type\":\"ConnectorPlacement.EquallySpacedRectSide\",\"uuid\":\"592cc1a1-656f-47ce-ad3a-4b4dc1070b5c\"},{\"content\":{\"connectorIds\":[\"RConn1\"],\"side\":\"RIGHT\"},\"type\":\"ConnectorPlacement.EquallySpacedRectSide\",\"uuid\":\"9bca39c3-eeb4-4456-9b97-61ec2f027d42\"},{\"content\":{\"connectorIds\":[],\"side\":\"TOP\"},\"type\":\"ConnectorPlacement.EquallySpacedRectSide\",\"uuid\":\"1e04bf27-fb0c-4be4-96d5-7a7c6152a7df\"},{\"content\":{\"connectorIds\":[\"Out1\"],\"side\":\"BOTTOM\"},\"type\":\"ConnectorPlacement.EquallySpacedRectSide\",\"uuid\":\"fcca2b0e-3afa-4320-884d-439bb49264b6\"}]},\"type\":\"ConnectorPlacement.EquallySpacedConnector\",\"uuid\":\"70eba8cc-e966-48e4-a1ce-5ccb9693dc60\"}],\"packageUris\":[\"http://schema.mathworks.com/mf0/Connector/R2020b\"],\"version\":\"1.0\"}"
      mask Display: disp('w');
  Sense wR1 : Subsystem
      settings: PortSchema="{\"entries\":[{\"content\":{\"sides\":[{\"content\":{\"connectorIds\":[\"LConn1\"]},\"type\":\"ConnectorPlacement.EquallySpacedRectSide\",\"uuid\":\"592cc1a1-656f-47ce-ad3a-4b4dc1070b5c\"},{\"content\":{\"connectorIds\":[\"RConn1\"],\"side\":\"RIGHT\"},\"type\":\"ConnectorPlacement.EquallySpacedRectSide\",\"uuid\":\"9bca39c3-eeb4-4456-9b97-61ec2f027d42\"},{\"content\":{\"connectorIds\":[],\"side\":\"TOP\"},\"type\":\"ConnectorPlacement.EquallySpacedRectSide\",\"uuid\":\"1e04bf27-fb0c-4be4-96d5-7a7c6152a7df\"},{\"content\":{\"connectorIds\":[\"Out1\"],\"side\":\"BOTTOM\"},\"type\":\"ConnectorPlacement.EquallySpacedRectSide\",\"uuid\":\"fcca2b0e-3afa-4320-884d-439bb49264b6\"}]},\"type\":\"ConnectorPlacement.EquallySpacedConnector\",\"uuid\":\"70eba8cc-e966-48e4-a1ce-5ccb9693dc60\"}],\"packageUris\":[\"http://schema.mathworks.com/mf0/Connector/R2020b\"],\"version\":\"1.0\"}"
      mask Display: disp('w');
  Sense wR2 : Subsystem
      settings: PortSchema="{\"entries\":[{\"content\":{\"sides\":[{\"content\":{\"connectorIds\":[\"LConn1\"]},\"type\":\"ConnectorPlacement.EquallySpacedRectSide\",\"uuid\":\"592cc1a1-656f-47ce-ad3a-4b4dc1070b5c\"},{\"content\":{\"connectorIds\":[\"RConn1\"],\"side\":\"RIGHT\"},\"type\":\"ConnectorPlacement.EquallySpacedRectSide\",\"uuid\":\"9bca39c3-eeb4-4456-9b97-61ec2f027d42\"},{\"content\":{\"connectorIds\":[],\"side\":\"TOP\"},\"type\":\"ConnectorPlacement.EquallySpacedRectSide\",\"uuid\":\"1e04bf27-fb0c-4be4-96d5-7a7c6152a7df\"},{\"content\":{\"connectorIds\":[\"Out1\"],\"side\":\"BOTTOM\"},\"type\":\"ConnectorPlacement.EquallySpacedRectSide\",\"uuid\":\"fcca2b0e-3afa-4320-884d-439bb49264b6\"}]},\"type\":\"ConnectorPlacement.EquallySpacedConnector\",\"uuid\":\"70eba8cc-e966-48e4-a1ce-5ccb9693dc60\"}],\"packageUris\":[\"http://schema.mathworks.com/mf0/Connector/R2020b\"],\"version\":\"1.0\"}"
      mask Display: disp('w');
  Sense wR3 : Subsystem
      settings: PortSchema="{\"entries\":[{\"content\":{\"sides\":[{\"content\":{\"connectorIds\":[\"LConn1\"]},\"type\":\"ConnectorPlacement.EquallySpacedRectSide\",\"uuid\":\"592cc1a1-656f-47ce-ad3a-4b4dc1070b5c\"},{\"content\":{\"connectorIds\":[\"RConn1\"],\"side\":\"RIGHT\"},\"type\":\"ConnectorPlacement.EquallySpacedRectSide\",\"uuid\":\"9bca39c3-eeb4-4456-9b97-61ec2f027d42\"},{\"content\":{\"connectorIds\":[],\"side\":\"TOP\"},\"type\":\"ConnectorPlacement.EquallySpacedRectSide\",\"uuid\":\"1e04bf27-fb0c-4be4-96d5-7a7c6152a7df\"},{\"content\":{\"connectorIds\":[\"Out1\"],\"side\":\"BOTTOM\"},\"type\":\"ConnectorPlacement.EquallySpacedRectSide\",\"uuid\":\"fcca2b0e-3afa-4320-884d-439bb49264b6\"}]},\"type\":\"ConnectorPlacement.EquallySpacedConnector\",\"uuid\":\"70eba8cc-e966-48e4-a1ce-5ccb9693dc60\"}],\"packageUris\":[\"http://schema.mathworks.com/mf0/Connector/R2020b\"],\"version\":\"1.0\"}"
      mask Display: disp('w');
  Simscape Bus1 : SimscapeBus  HierarchyStrings=L1;L2;L3;R1;R2;R3
  Simulink-PS Converter{,4,7..9} (5 alike) : nesl_utility/Simulink-PS Converter  PhysicalDomain=network_engine_domain  SubClassName=ps_input  LeftPortType=input  RightPortType=output  PseudoPeriodic=off  Frequencies=[]  NoiseDistribution=none  NoiseParameters=[]  Unit=1  AffineConversion=off  FilteringAndDerivatives=provide  SimscapeFilterOrder=1  InputFilterTimeConstant=0.001  UdotUserProvided=0
  Simulink-PS Converter5 : nesl_utility/Simulink-PS Converter  PhysicalDomain=network_engine_domain  SubClassName=ps_input  LeftPortType=input  RightPortType=output  PseudoPeriodic=off  Frequencies=[]  NoiseDistribution=none  NoiseParameters=[]  Unit=1  AffineConversion=off  FilteringAndDerivatives=zero  SimscapeFilterOrder=2  InputFilterTimeConstant=0.001  UdotUserProvided=0
  Torque Source L1 : fl_lib/Mechanical/Mechanical Sources/Ideal Torque Source
  Torque Source L2 : fl_lib/Mechanical/Mechanical Sources/Ideal Torque Source
  Torque Source L3 : fl_lib/Mechanical/Mechanical Sources/Ideal Torque Source
  Torque Source R1 : fl_lib/Mechanical/Mechanical Sources/Ideal Torque Source
  Torque Source R2 : fl_lib/Mechanical/Mechanical Sources/Ideal Torque Source
  Torque Source R3 : fl_lib/Mechanical/Mechanical Sources/Ideal Torque Source
  Transfer Fcn{,1..5} (6 alike) : TransferFcn  Denominator=[motor_tc 1]
  C : PMIOPort  Side=Left
  S : PMIOPort  Port=2  Side=Right
  Out Bus Element : Outport  PortName=m  Element=trq.L1
  Out Bus Element1 : Outport  PortName=m  Element=trq.L2
  Out Bus Element2 : Outport  PortName=m  Element=trq.L3
  Out Bus Element3 : Outport  PortName=m  Element=trq.R1
  Out Bus Element4 : Outport  PortName=m  Element=trq.R2
  Out Bus Element5 : Outport  PortName=m  Element=trq.R3
  Out Bus Element6 : Outport  PortName=m  Element=w.L1
  Out Bus Element7 : Outport  PortName=m  Element=w.L2
  Out Bus Element8 : Outport  PortName=m  Element=w.L3
  Out Bus Element9 : Outport  PortName=m  Element=w.R1
  Out Bus Element10 : Outport  PortName=m  Element=w.R2
  Out Bus Element11 : Outport  PortName=m  Element=w.R3
  wires:
  Gain3/1 -> Out Bus Element3/1, Simulink-PS Converter5/1
  Gain4/1 -> Out Bus Element4/1, Simulink-PS Converter9/1
  Gain5/1 -> Out Bus Element5/1, Simulink-PS Converter4/1
  Gain/1 -> Out Bus Element/1, Simulink-PS Converter8/1
  Gain1/1 -> Out Bus Element1/1, Simulink-PS Converter7/1
  Gain2/1 -> Simulink-PS Converter/1, Out Bus Element2/1
  Sense wL1/1(w) -> Out Bus Element6/1
  Sense wL2/1(w) -> Out Bus Element7/1
  Sense wL3/1(w) -> Out Bus Element8/1
  Sense wR1/1(w) -> Out Bus Element9/1
  Sense wR2/1(w) -> Out Bus Element10/1
  Sense wR3/1(w) -> Out Bus Element11/1
  In Bus Element8/1 -> Transfer Fcn/1
  Transfer Fcn/1 -> Gain2/1
  Transfer Fcn1/1 -> Gain1/1
  In Bus Element7/1 -> Transfer Fcn1/1
  In Bus Element6/1 -> Transfer Fcn2/1
  Transfer Fcn2/1 -> Gain/1
  Transfer Fcn3/1 -> Gain5/1
  In Bus Element11/1 -> Transfer Fcn3/1
  In Bus Element10/1 -> Transfer Fcn4/1
  Transfer Fcn4/1 -> Gain4/1
  Transfer Fcn5/1 -> Gain3/1
  In Bus Element9/1 -> Transfer Fcn5/1
  connections:
  Torque Source L1/RConn1 -- Simulink-PS Converter8/RConn1
  Gear R3/RConn1 -- Connection Label17/LConn1
  Torque Source L3/RConn2 -- Sense wL3/LConn1 -- Damper L3/RConn1 -- Sense wL2/LConn1 -- Damper L2/RConn1 -- Torque Source L2/RConn2 -- Damper L1/RConn1 -- Sense wL1/LConn1 -- Torque Source L1/RConn2 -- C/RConn1 -- Damper R2/RConn1 -- Sense wR2/LConn1 -- Torque Source R2/RConn2 -- Sense wR1/LConn1 -- Damper R1/RConn1 -- Torque Source R1/RConn2 -- Damper R3/RConn1 -- Sense wR3/LConn1 -- Torque Source R3/RConn2
  Gear R2/RConn1 -- Connection Label12/LConn1
  Simulink-PS Converter7/RConn1 -- Torque Source L2/RConn1
  Torque Source R1/RConn1 -- Simulink-PS Converter5/RConn1
  Gear L1/RConn1 -- Connection Label2/LConn1
  Simulink-PS Converter9/RConn1 -- Torque Source R2/RConn1
  Gear L2/RConn1 -- Connection Label4/LConn1
  Simulink-PS Converter4/RConn1 -- Torque Source R3/RConn1
  Gear L3/RConn1 -- Connection Label19/LConn1
  Simulink-PS Converter/RConn1 -- Torque Source L3/RConn1
  Simscape Bus1/LConn4 -- Connection Label15/LConn1
  Simscape Bus1/LConn2 -- Connection Label25/LConn1
  Simscape Bus1/LConn6 -- Connection Label20/LConn1
  Simscape Bus1/LConn3 -- Connection Label28/LConn1
  Simscape Bus1/LConn1 -- Connection Label23/LConn1
  Simscape Bus1/LConn5 -- Connection Label16/LConn1
  Simscape Bus1/RConn1 -- S/RConn1
  Gear L1/LConn1 -- Sense wL1/RConn1 -- Damper L1/LConn1 -- Torque Source L1/LConn1
  Gear L2/LConn1 -- Sense wL2/RConn1 -- Damper L2/LConn1 -- Torque Source L2/LConn1
  Gear L3/LConn1 -- Sense wL3/RConn1 -- Damper L3/LConn1 -- Torque Source L3/LConn1
  Torque Source R1/LConn1 -- Sense wR1/RConn1 -- Damper R1/LConn1 -- Gear R1/LConn1
  Gear R1/RConn1 -- Connection Label11/LConn1
  Gear R2/LConn1 -- Sense wR2/RConn1 -- Damper R2/LConn1 -- Torque Source R2/LConn1
  Gear R3/LConn1 -- Damper R3/LConn1 -- Sense wR3/RConn1 -- Torque Source R3/LConn1
